simulink model "RC_model"  (R2024b)
settings: Solver=VariableStepAuto  StartTime=0.0  StopTime=3531.05  MaxStep=0.05  RelTol=1e-3
values from neighbouring files (symbols this model uses):
  R1 = 100    [Parameter_fitting_with_saving.m]    (also in Simulating_with_fixed_parameters.m = 889.625; initialization.m = 0.015)
  R2 = 100    [Parameter_fitting_with_saving.m]    (also in initialization.m = 0.02)
  R3 = 100    [Parameter_fitting_with_saving.m]    (also in initialization.m = 0.03)
  R_leak = 800    [Parameter_fitting_with_saving.m]    (also in Simulating_with_fixed_parameters.m = 1000.16; initialization.m = 0.001)
  R_s = 7.6e-3*5    (= 0.038)    [Parameter_fitting_with_saving.m]    (also in Simulating_with_fixed_parameters.m; initialization.m = 0.15)
  V_initial = voltage(1)    [Parameter_fitting_with_saving.m]    (also in Simulating_with_fixed_parameters.m)
undefined symbols (not defined in the file or in its folder): Ini_fac1, Ini_fac2, Ini_fac3
libraries: fl_lib x112, nesl_utility x57, ee_lib x2
(part 2 of 2)

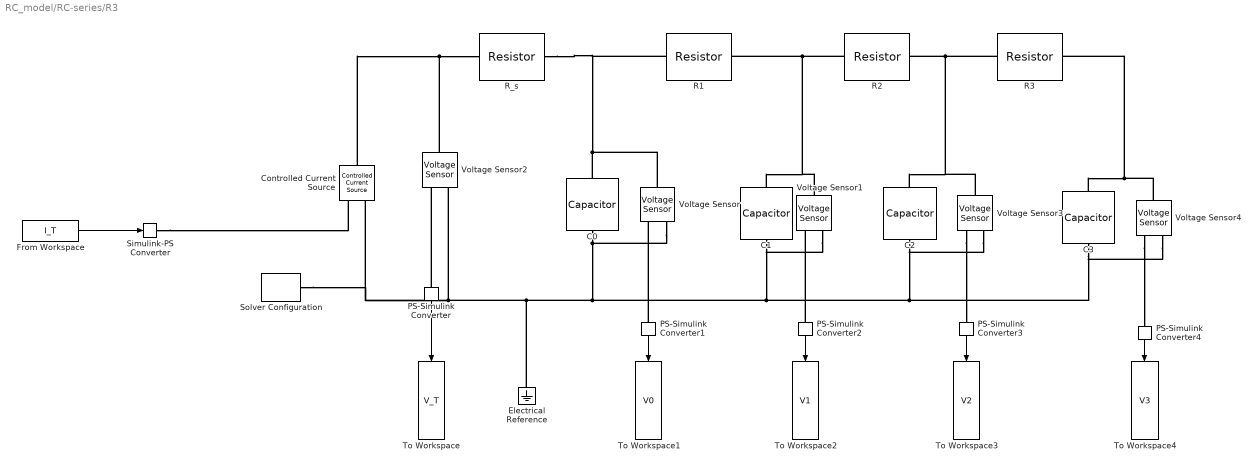
== system RC_model/RC-series/R3 ==
  C0 : fl_lib/Electrical/Electrical Elements/Capacitor  c=C0 F  r=0 Ohm  g=0 1/Ohm  i_specify=off  i_priority=None  i=0 A  i_nominal_specify=off  i_nominal_value=1  i_nominal_unit=A  v_specify=off  v_priority=None  v=0 V  v_nominal_specify=off  v_nominal_value=1  v_nominal_unit=V  vc_specify=on  vc_priority=High  vc=V_initial*Ini_fac1 V  vc_nominal_specify=off  vc_nominal_value=1  vc_nominal_unit=V
  C1 : fl_lib/Electrical/Electrical Elements/Capacitor  c=C1 F  r=0 Ohm  g=0 1/Ohm  i_specify=off  i_priority=None  i=0 A  i_nominal_specify=off  i_nominal_value=1  i_nominal_unit=A  v_specify=off  v_priority=None  v=0 V  v_nominal_specify=off  v_nominal_value=1  v_nominal_unit=V  vc_specify=on  vc_priority=Low  vc=V_initial*Ini_fac2 V  vc_nominal_specify=off  vc_nominal_value=1  vc_nominal_unit=V
  C2 : fl_lib/Electrical/Electrical Elements/Capacitor  c=C2 F  r=0 Ohm  g=0 1/Ohm  i_specify=off  i_priority=None  i=0 A  i_nominal_specify=off  i_nominal_value=1  i_nominal_unit=A  v_specify=off  v_priority=None  v=0 V  v_nominal_specify=off  v_nominal_value=1  v_nominal_unit=V  vc_specify=on  vc_priority=Low  vc=V_initial*Ini_fac3 V  vc_nominal_specify=off  vc_nominal_value=1  vc_nominal_unit=V
  C3 : fl_lib/Electrical/Electrical Elements/Capacitor  c=C3 F  r=0 Ohm  g=0 1/Ohm  i_specify=off  i_priority=None  i=0 A  i_nominal_specify=off  i_nominal_value=1  i_nominal_unit=A  v_specify=off  v_priority=None  v=0 V  v_nominal_specify=off  v_nominal_value=1  v_nominal_unit=V  vc_specify=on  vc_priority=Low  vc=V_initial*Ini_fac3 V  vc_nominal_specify=off  vc_nominal_value=1  vc_nominal_unit=V
  Controlled Current Source : fl_lib/Electrical/Electrical Sources/Controlled Current Source
  Electrical Reference : fl_lib/Electrical/Electrical Elements/Electrical Reference
  From Workspace : FromWorkspace  VariableName=I_T
  PS-Simulink Converter{,1..4} (5 alike) : nesl_utility/PS-Simulink Converter  PhysicalDomain=network_engine_domain  SubClassName=ps_output  LeftPortType=input  RightPortType=output  PseudoPeriodic=off  Frequencies=[]  VectorFormat=inherit  Unit=inherit  AffineConversion=off
  R1 : fl_lib/Electrical/Electrical Elements/Resistor  R=R1 Ohm  i_specify=off  i_priority=None  i=0 A  i_nominal_specify=off  i_nominal_value=1  i_nominal_unit=A  v_specify=off  v_priority=None  v=0 V  v_nominal_specify=off  v_nominal_value=1  v_nominal_unit=V
  R2 : fl_lib/Electrical/Electrical Elements/Resistor  R=R2 Ohm  i_specify=off  i_priority=None  i=0 A  i_nominal_specify=off  i_nominal_value=1  i_nominal_unit=A  v_specify=off  v_priority=None  v=0 V  v_nominal_specify=off  v_nominal_value=1  v_nominal_unit=V
  R3 : fl_lib/Electrical/Electrical Elements/Resistor  R=R3 Ohm  i_specify=off  i_priority=None  i=0 A  i_nominal_specify=off  i_nominal_value=1  i_nominal_unit=A  v_specify=off  v_priority=None  v=0 V  v_nominal_specify=off  v_nominal_value=1  v_nominal_unit=V
  R_s : fl_lib/Electrical/Electrical Elements/Resistor  R=R_s Ohm  i_specify=off  i_priority=None  i=0 A  i_nominal_specify=off  i_nominal_value=1  i_nominal_unit=A  v_specify=off  v_priority=None  v=0 V  v_nominal_specify=off  v_nominal_value=1  v_nominal_unit=V
  Simulink-PS Converter : nesl_utility/Simulink-PS Converter  PhysicalDomain=network_engine_domain  SubClassName=ps_input  LeftPortType=input  RightPortType=output  PseudoPeriodic=off  Frequencies=[]  NoiseDistribution=none  NoiseParameters=[]  Unit=1  AffineConversion=off  FilteringAndDerivatives=provide  SimscapeFilterOrder=1  InputFilterTimeConstant=0.001  UdotUserProvided=0
  Solver Configuration : nesl_utility/Solver Configuration  PhysicalDomain=network_engine_domain  SubClassName=solver  LeftPortType=input  RightPortType=generic  Tones=[]  Harmonics=[]  SimulateNoise=off  Profile=off  UseLocalSampling=off  EnableSwitchedLinearOptims=on  FrequencyDomain=off  UseCCode=off  RelTol=0.001  AbsTol=0.001  MinStep=1e-09  ToWorkspace=off  RevertToSquareIcSolve=off  NumHomotopyIterations=100  PhasorMode=off  PhasorModeNumHarmonics=1  ConsistencySolver=NEWTON_XTOL_AFTER_FTOL  IndexReductionMethod=DerivativeReplacement  DoDC=off  ResidualTolerance=1e-09  ConsistencyTolSource=GLOBAL  ConsistencyAbsTol=0.001  ConsistencyRelTol=0.001  ConsistencyTolFactor=0.001  UseLocalSolver=off  LocalSolverChoice=NE_BACKWARD_EULER_ADVANCER  ResolveIndetEquations=on  FunctionEvalNumThread=1  LocalSolverSampleTime=0.001  DoFixedCost=off  MaxNonlinIter=3  MaxModeIter=2  ComputeImpulses=off  ImpulseIterations=2  LinearAlgebra=auto  LinearAlgebraNumThread=0  EquationFormulation=NE_TIME_EF  DelaysMemoryBudget=1024  AutomaticFiltering=on  FilteringTimeConstant=0.001  PartitionStorageMethod=AS_NEEDED  PartitionMemoryBudget=1024  PartitionMethod=ROBUST  MultibodyUseLocalSolver=off  MultibodyLocalSolverChoice=ODE1  MultibodyLocalSolverSampleTime=0.001
  To Workspace : ToWorkspace  VariableName=V_T  SaveFormat=Timeseries  SampleTime=-1
  To Workspace1 : ToWorkspace  VariableName=V0  SaveFormat=Timeseries  SampleTime=-1
  To Workspace2 : ToWorkspace  VariableName=V1  SaveFormat=Timeseries  SampleTime=-1
  To Workspace3 : ToWorkspace  VariableName=V2  SaveFormat=Timeseries  SampleTime=-1
  To Workspace4 : ToWorkspace  VariableName=V3  SaveFormat=Timeseries  SampleTime=-1
  Voltage Sensor{,1..4} (5 alike) : fl_lib/Electrical/Electrical Sensors/Voltage Sensor
  wires:
  PS-Simulink Converter/1 -> To Workspace/1
  PS-Simulink Converter2/1 -> To Workspace2/1
  PS-Simulink Converter1/1 -> To Workspace1/1
  PS-Simulink Converter3/1 -> To Workspace3/1
  PS-Simulink Converter4/1 -> To Workspace4/1
  From Workspace/1 -> Simulink-PS Converter/1
  connections:
  C0/LConn1 -- R1/LConn1 -- R_s/RConn1 -- Voltage Sensor/LConn1
  Voltage Sensor/RConn2 -- C0/RConn1 -- Electrical Reference/LConn1 -- Controlled Current Source/RConn2 -- Solver Configuration/RConn1 -- Voltage Sensor2/RConn2 -- Voltage Sensor1/RConn2 -- C1/RConn1 -- Voltage Sensor3/RConn2 -- C2/RConn1 -- C3/RConn1 -- Voltage Sensor4/RConn2
  Voltage Sensor2/LConn1 -- Controlled Current Source/LConn1 -- R_s/LConn1
  C1/LConn1 -- Voltage Sensor1/LConn1 -- R2/LConn1 -- R1/RConn1
  PS-Simulink Converter/LConn1 -- Voltage Sensor2/RConn1
  PS-Simulink Converter1/LConn1 -- Voltage Sensor/RConn1
  C2/LConn1 -- Voltage Sensor3/LConn1 -- R2/RConn1 -- R3/LConn1
  Voltage Sensor3/RConn1 -- PS-Simulink Converter3/LConn1
  PS-Simulink Converter2/LConn1 -- Voltage Sensor1/RConn1
  C3/LConn1 -- Voltage Sensor4/LConn1 -- R3/RConn1
  Voltage Sensor4/RConn1 -- PS-Simulink Converter4/LConn1
  Simulink-PS Converter/RConn1 -- Controlled Current Source/RConn1

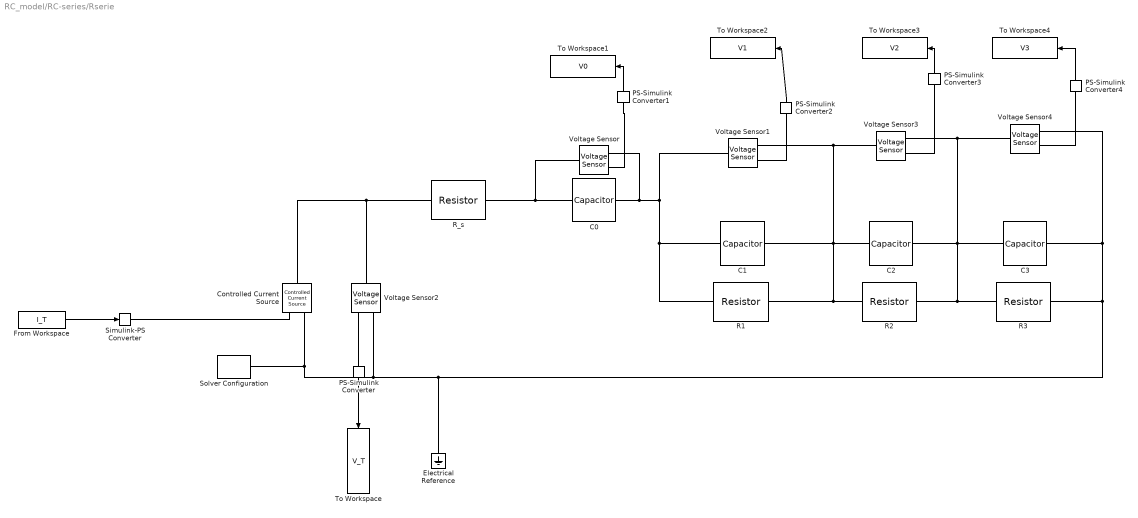
== system RC_model/RC-series/Rserie ==
  C0 : fl_lib/Electrical/Electrical Elements/Capacitor  c=C0 F  r=0 Ohm  g=0 1/Ohm  i_specify=off  i_priority=None  i=0 A  i_nominal_specify=off  i_nominal_value=1  i_nominal_unit=A  v_specify=off  v_priority=None  v=0 V  v_nominal_specify=off  v_nominal_value=1  v_nominal_unit=V  vc_specify=on  vc_priority=High  vc=V_initial V  vc_nominal_specify=off  vc_nominal_value=1  vc_nominal_unit=V
  C1 : fl_lib/Electrical/Electrical Elements/Capacitor  c=C1 F  r=0 Ohm  g=0 1/Ohm  i_specify=off  i_priority=None  i=0 A  i_nominal_specify=off  i_nominal_value=1  i_nominal_unit=A  v_specify=off  v_priority=None  v=0 V  v_nominal_specify=off  v_nominal_value=1  v_nominal_unit=V  vc_specify=on  vc_priority=None  vc=V_initial V  vc_nominal_specify=off  vc_nominal_value=1  vc_nominal_unit=V
  C2 : fl_lib/Electrical/Electrical Elements/Capacitor  c=C2 F  r=0 Ohm  g=0 1/Ohm  i_specify=off  i_priority=None  i=0 A  i_nominal_specify=off  i_nominal_value=1  i_nominal_unit=A  v_specify=off  v_priority=None  v=0 V  v_nominal_specify=off  v_nominal_value=1  v_nominal_unit=V  vc_specify=on  vc_priority=None  vc=V_initial V  vc_nominal_specify=off  vc_nominal_value=1  vc_nominal_unit=V
  C3 : fl_lib/Electrical/Electrical Elements/Capacitor  c=C3 F  r=0 Ohm  g=0 1/Ohm  i_specify=off  i_priority=None  i=0 A  i_nominal_specify=off  i_nominal_value=1  i_nominal_unit=A  v_specify=off  v_priority=None  v=0 V  v_nominal_specify=off  v_nominal_value=1  v_nominal_unit=V  vc_specify=on  vc_priority=None  vc=V_initial V  vc_nominal_specify=off  vc_nominal_value=1  vc_nominal_unit=V
  Controlled Current Source : fl_lib/Electrical/Electrical Sources/Controlled Current Source
  Electrical Reference : fl_lib/Electrical/Electrical Elements/Electrical Reference
  From Workspace : FromWorkspace  VariableName=I_T
  PS-Simulink Converter{,1..4} (5 alike) : nesl_utility/PS-Simulink Converter  PhysicalDomain=network_engine_domain  SubClassName=ps_output  LeftPortType=input  RightPortType=output  PseudoPeriodic=off  Frequencies=[]  VectorFormat=inherit  Unit=inherit  AffineConversion=off
  R1 : fl_lib/Electrical/Electrical Elements/Resistor  R=R1 Ohm  i_specify=off  i_priority=None  i=0 A  i_nominal_specify=off  i_nominal_value=1  i_nominal_unit=A  v_specify=off  v_priority=None  v=0 V  v_nominal_specify=off  v_nominal_value=1  v_nominal_unit=V
  R2 : fl_lib/Electrical/Electrical Elements/Resistor  R=R2 Ohm  i_specify=off  i_priority=None  i=0 A  i_nominal_specify=off  i_nominal_value=1  i_nominal_unit=A  v_specify=off  v_priority=None  v=0 V  v_nominal_specify=off  v_nominal_value=1  v_nominal_unit=V
  R3 : fl_lib/Electrical/Electrical Elements/Resistor  R=R3 Ohm  i_specify=off  i_priority=None  i=0 A  i_nominal_specify=off  i_nominal_value=1  i_nominal_unit=A  v_specify=off  v_priority=None  v=0 V  v_nominal_specify=off  v_nominal_value=1  v_nominal_unit=V
  R_s : fl_lib/Electrical/Electrical Elements/Resistor  R=R_s Ohm  i_specify=off  i_priority=None  i=0 A  i_nominal_specify=off  i_nominal_value=1  i_nominal_unit=A  v_specify=off  v_priority=None  v=0 V  v_nominal_specify=off  v_nominal_value=1  v_nominal_unit=V
  Simulink-PS Converter : nesl_utility/Simulink-PS Converter  PhysicalDomain=network_engine_domain  SubClassName=ps_input  LeftPortType=input  RightPortType=output  PseudoPeriodic=off  Frequencies=[]  NoiseDistribution=none  NoiseParameters=[]  Unit=1  AffineConversion=off  FilteringAndDerivatives=provide  SimscapeFilterOrder=1  InputFilterTimeConstant=0.001  UdotUserProvided=0
  Solver Configuration : nesl_utility/Solver Configuration  PhysicalDomain=network_engine_domain  SubClassName=solver  LeftPortType=input  RightPortType=generic  Tones=[]  Harmonics=[]  SimulateNoise=off  Profile=off  UseLocalSampling=off  EnableSwitchedLinearOptims=on  FrequencyDomain=off  UseCCode=off  RelTol=0.001  AbsTol=0.001  MinStep=1e-09  ToWorkspace=off  RevertToSquareIcSolve=off  NumHomotopyIterations=100  PhasorMode=off  PhasorModeNumHarmonics=1  ConsistencySolver=NEWTON_XTOL_AFTER_FTOL  IndexReductionMethod=DerivativeReplacement  DoDC=off  ResidualTolerance=1e-09  ConsistencyTolSource=GLOBAL  ConsistencyAbsTol=0.001  ConsistencyRelTol=0.001  ConsistencyTolFactor=0.001  UseLocalSolver=off  LocalSolverChoice=NE_BACKWARD_EULER_ADVANCER  ResolveIndetEquations=on  FunctionEvalNumThread=1  LocalSolverSampleTime=0.001  DoFixedCost=off  MaxNonlinIter=3  MaxModeIter=2  ComputeImpulses=off  ImpulseIterations=2  LinearAlgebra=auto  LinearAlgebraNumThread=0  EquationFormulation=NE_TIME_EF  DelaysMemoryBudget=1024  AutomaticFiltering=on  FilteringTimeConstant=0.001  PartitionStorageMethod=AS_NEEDED  PartitionMemoryBudget=1024  PartitionMethod=ROBUST  MultibodyUseLocalSolver=off  MultibodyLocalSolverChoice=ODE1  MultibodyLocalSolverSampleTime=0.001
  To Workspace : ToWorkspace  VariableName=V_T  SaveFormat=Timeseries  SampleTime=-1
  To Workspace1 : ToWorkspace  VariableName=V0  SaveFormat=Timeseries  SampleTime=-1
  To Workspace2 : ToWorkspace  VariableName=V1  SaveFormat=Timeseries  SampleTime=-1
  To Workspace3 : ToWorkspace  VariableName=V2  SaveFormat=Timeseries  SampleTime=-1
  To Workspace4 : ToWorkspace  VariableName=V3  SaveFormat=Timeseries  SampleTime=-1
  Voltage Sensor{,1..4} (5 alike) : fl_lib/Electrical/Electrical Sensors/Voltage Sensor
  wires:
  PS-Simulink Converter/1 -> To Workspace/1
  PS-Simulink Converter2/1 -> To Workspace2/1
  PS-Simulink Converter1/1 -> To Workspace1/1
  PS-Simulink Converter3/1 -> To Workspace3/1
  PS-Simulink Converter4/1 -> To Workspace4/1
  From Workspace/1 -> Simulink-PS Converter/1
  connections:
  R1/LConn1 -- Voltage Sensor1/LConn1 -- C0/RConn1 -- Voltage Sensor/RConn2 -- C1/LConn1
  C3/RConn1 -- Voltage Sensor4/RConn2 -- Electrical Reference/LConn1 -- Voltage Sensor2/RConn2 -- Controlled Current Source/RConn2 -- Solver Configuration/RConn1 -- R3/RConn1
  Voltage Sensor/LConn1 -- R_s/RConn1 -- C0/LConn1
  R2/LConn1 -- C1/RConn1 -- Voltage Sensor1/RConn2 -- Voltage Sensor3/LConn1 -- C2/LConn1 -- R1/RConn1
  PS-Simulink Converter/LConn1 -- Voltage Sensor2/RConn1
  PS-Simulink Converter1/LConn1 -- Voltage Sensor/RConn1
  R3/LConn1 -- C2/RConn1 -- Voltage Sensor4/LConn1 -- Voltage Sensor3/RConn2 -- C3/LConn1 -- R2/RConn1
  Voltage Sensor3/RConn1 -- PS-Simulink Converter3/LConn1
  Voltage Sensor4/RConn1 -- PS-Simulink Converter4/LConn1
  Simulink-PS Converter/RConn1 -- Controlled Current Source/RConn1
  Voltage Sensor1/RConn1 -- PS-Simulink Converter2/LConn1
  Controlled Current Source/LConn1 -- R_s/LConn1 -- Voltage Sensor2/LConn1
